simulink model "fir_fsm"  (R2026a)
settings: Solver=FixedStepDiscrete  StopTime=300  FixedStep=1
model workspace (MAT data in the model file):
  b = [0.125 0.375 0.375 0.125]
  f_noise = 0.4
  f_sig = 0.01
settings Model: Creator=KoayXianCong  LastModifiedBy=KoayXianCong

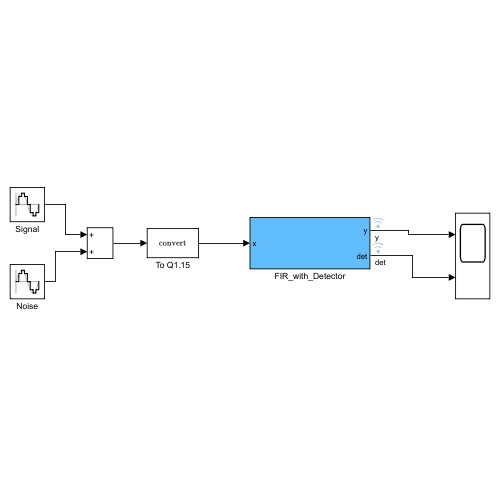
[thumbnail: Simulink's stored preview of the top-level diagram]
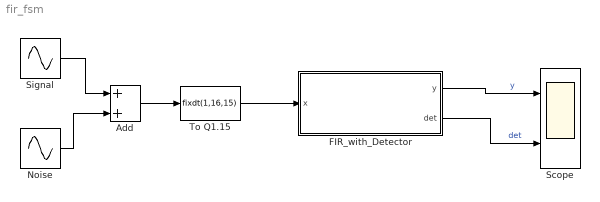
== system fir_fsm ==
  Add : Sum
  FIR_with_Detector : Subsystem
  Noise : Sin  Amplitude=0.4  Frequency=2*pi*f_noise  SampleTime=1
  Scope : Scope  NumInputPorts=2
      settings: TimeSpan=300
  Signal : Sin  Amplitude=0.5  Frequency=2*pi*f_sig  SampleTime=1
  To Q1.15 : DataTypeConversion  OutDataTypeStr=fixdt(1,16,15)  RndMeth=Nearest
  wires:
  Signal/1 -> Add/1
  Noise/1 -> Add/2
  Add/1 -> To Q1.15/1
  To Q1.15/1 -> FIR_with_Detector/1(x)
  FIR_with_Detector/1(y) -> Scope/1  "y"
  FIR_with_Detector/2(det) -> Scope/2  "det"

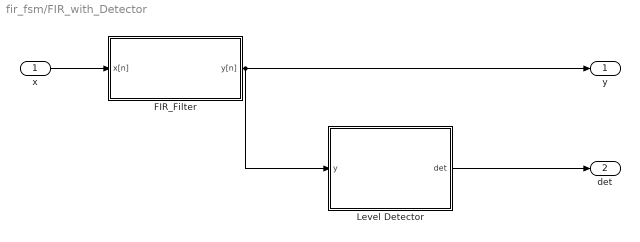
== system fir_fsm/FIR_with_Detector ==
  x : Inport
  FIR_Filter : Subsystem
  Level Detector : Stateflow chart  TreatAsAtomicUnit=on
  y : Outport
  det : Outport  Port=2
  wires:
  x/1 -> FIR_Filter/1(x[n])
  FIR_Filter/1(y[n]) -> y/1, Level Detector/1(y)
  Level Detector/1(det) -> det/1

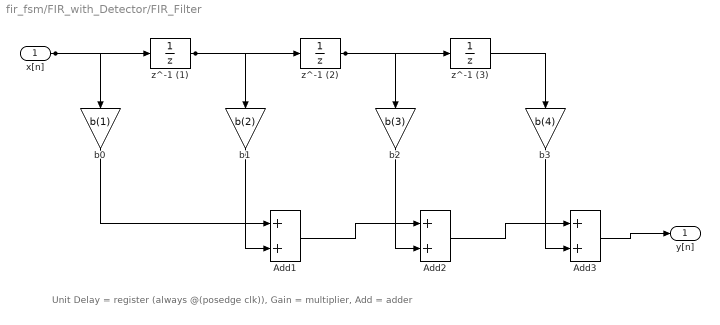
== system fir_fsm/FIR_with_Detector/FIR_Filter ==
  note: Unit Delay = register (always @(posedge clk)), Gain = multiplier, Add = adder
  x[n] : Inport
  Add1 : Sum  OutDataTypeStr=fixdt(1,19,18)
  Add2 : Sum  OutDataTypeStr=fixdt(1,19,18)
  Add3 : Sum  OutDataTypeStr=fixdt(1,19,18)
  b0 : Gain  Gain=b(1)  ParamDataTypeStr=fixdt(1,16,15)  OutDataTypeStr=fixdt(1,19,18)
  b1 : Gain  Gain=b(2)  ParamDataTypeStr=fixdt(1,16,15)  OutDataTypeStr=fixdt(1,19,18)
  b2 : Gain  Gain=b(3)  ParamDataTypeStr=fixdt(1,16,15)  OutDataTypeStr=fixdt(1,19,18)
  b3 : Gain  Gain=b(4)  ParamDataTypeStr=fixdt(1,16,15)  OutDataTypeStr=fixdt(1,19,18)
  z^-1 (1) : UnitDelay  SampleTime=-1
  z^-1 (2) : UnitDelay  SampleTime=-1
  z^-1 (3) : UnitDelay  SampleTime=-1
  y[n] : Outport
  wires:
  Add3/1 -> y[n]/1
  b3/1 -> Add3/2
  Add2/1 -> Add3/1
  b2/1 -> Add2/2
  Add1/1 -> Add2/1
  b1/1 -> Add1/2
  b0/1 -> Add1/1
  z^-1 (3)/1 -> b3/1
  z^-1 (2)/1 -> b2/1, z^-1 (3)/1
  z^-1 (1)/1 -> b1/1, z^-1 (2)/1
  x[n]/1 -> b0/1, z^-1 (1)/1

== stateflow chart fir_fsm/FIR_with_Detector/Level Detector ==
  state LOW
    entry: det = false;
  state ARM_HI
    entry: cnt = uint8(0);
    during: cnt = cnt + 1;
  state ARM_LO
    entry: cnt = uint8(0);
    during: cnt = cnt + 1;
  state HIGH
    entry: det = true;
  (default) -> LOW
  LOW -> ARM_HI : [y > TH]
  ARM_HI -> LOW [order 1] : [y <= TH]
  ARM_LO -> LOW [order 2] : [cnt >= N]
  ARM_HI -> HIGH [order 2] : [cnt >= N]
  ARM_LO -> HIGH [order 1] : [y >= TH]
  HIGH -> ARM_LO : [y < TH]
  data: y input; det output boolean; cnt local uint8; TH constant fixdt(1,19,18) =0.25; N constant uint8 =3
